simulink model "s_b4a4x1kf"  (R2018a)
settings: Solver=VariableStepDiscrete  StartTime=0.0  StopTime=1  RelTol=1e-3
undefined symbols (not defined in the file): fft_stages, n_bits_ants, n_bits_xengs
libraries: xbsIndex_r4 x22055, xbsReplacements_r4 x30, casper_library_misc x29, casper_library_scopes x15, xps_library x4
(part 29 of 227)

== system s_b4a4x1kf/sys1/vacc_tvg0 ==
  note: This counter increments by
      | one per accumulation.
      | Might be buggy; not tested.
  note: this TVG injects the same
      | number for vector_len.
      | Increments on vector edge.
      | (ramp over time)
  note: this TVG increments on
      | each valid input and resets
      | on vector_edge.
      | (ramp over channels).
  sync_in : Inport
  valid_in : Inport  Port=2
  data_in : Inport  Port=3
  time_in : Inport  Port=4
  acc_start_time : Inport  Port=5
  acc_len : Inport  Port=6
  Delay{,2..8} (8 alike) : xbsIndex_r4/Delay  rst=off  infoeditControl=Selection of Reset will increase slice count due to use of real FFs and instead of SRLs  en=off  latency=1  reg_retiming=on  dbl_ovrd=off  block_type=delay
      Delay settings: xl_area=[0, 0, 0, 0, 0, 0, 0]
      Delay2 settings: infoedit=Hardware notes: A delay line is a chain, each link of which is an SRL16 or SRL32 followed by a flip-flop.  xl_area=[0, 0, 0, 0, 0, 0, 0]
  Delay1 : xbsIndex_r4/Delay  rst=off  infoeditControl=Selection of Reset will increase slice count due to use of real FFs and instead of SRLs  en=off  latency=2  reg_retiming=on  dbl_ovrd=off  block_type=delay
      settings: infoedit=Hardware notes: A delay line is a chain, each link of which is an SRL16 or SRL32 followed by a flip-flop.  xl_area=[0, 0, 0, 0, 0, 0, 0]
  Delay9 : xbsIndex_r4/Delay  rst=off  infoeditControl=Selection of Reset will increase slice count due to use of real FFs and instead of SRLs  en=off  latency=3  reg_retiming=on  dbl_ovrd=off  block_type=delay
      settings: infoedit=Hardware notes: A delay line is a chain, each link of which is an SRL16 or SRL32 followed by a flip-flop.
  Mux1 : xbsIndex_r4/Mux  inputs=2  en=off  latency=1  precision=Full  arith_type="Signed  (2's comp)"  n_bits=8  bin_pt=2  quantization=Truncate  overflow=Wrap  dbl_ovrd=off  block_type=mux
      settings: xl_area=[0, 0, 0, 0, 0, 0, 0]
  Mux2 : xbsIndex_r4/Mux  inputs=2  en=off  latency=1  precision=Full  arith_type="Signed  (2's comp)"  n_bits=8  bin_pt=2  quantization=Truncate  overflow=Wrap  dbl_ovrd=off  block_type=mux
      settings: xl_area=[0, 0, 0, 0, 0, 0, 0]
  Mux3 : xbsIndex_r4/Mux  inputs=2  en=off  latency=1  precision=Full  arith_type="Signed  (2's comp)"  n_bits=8  bin_pt=2  quantization=Truncate  overflow=Wrap  dbl_ovrd=off  block_type=mux
      settings: xl_area=[0, 0, 0, 0, 0, 0, 0]
  Pulse Generator3 : DiscretePulseGenerator  Amplitude=25  Period=99999999  PulseWidth=500000  PhaseDelay=450000
  Relational2 : xbsIndex_r4/Relational  mode=a=b  op_type=Bool  en=off  latency=1  dbl_ovrd=off  block_type=relational
      settings: block_version=10.1.3
  Slice8 : xbsIndex_r4/Slice  nbits=n_bits  boolean_output=off  mode=Lower Bit Location + Width  bit1=0  base1=MSB of Input  bit0=0  base0=LSB of Input  dbl_ovrd=off  block_type=slice
  Slice9 : xbsIndex_r4/Slice  nbits=n_bits  boolean_output=off  mode=Lower Bit Location + Width  bit1=0  base1=MSB of Input  bit0=0  base0=LSB of Input  dbl_ovrd=off  block_type=slice
  Terminator5 : Terminator
  bus_replicate1 : Subsystem  Tag=cmac_delinked  mask(bus_replicate){replication=n_inputs, csp_latency=0, misc=off, implementation=core}
      mask prompts: replication "replication factor"; csp_latency "latency"; misc "misc support"; implementation "delay implementation"
      mask help: Output bus formed by replicating input bus a number of times
      mask init:
      | bus_replicate_init(gcb, ...
      |     'replication', replication, ...
      |     'csp_latency', csp_latency, ...
      |     'implementation', implementation, ...
      |     'misc', misc);
      mask TypeOptions implementation: core | behavioral
  bus_replicate2 : Subsystem  Tag=cmac_delinked  mask(bus_replicate){replication=n_inputs, csp_latency=0, misc=off, implementation=core}
      mask prompts: replication "replication factor"; csp_latency "latency"; misc "misc support"; implementation "delay implementation"
      mask help: Output bus formed by replicating input bus a number of times
      mask init:
      | bus_replicate_init(gcb, ...
      |     'replication', replication, ...
      |     'csp_latency', csp_latency, ...
      |     'implementation', implementation, ...
      |     'misc', misc);
      mask TypeOptions implementation: core | behavioral
  edge_detect : Subsystem  mask(edge_detect){edge=Rising, polarity=Active High, x_in=[0 0.08 0.08 0.16 0.16 0.24 0.24 0.32 0.32 0.4], y_in=[-1 -1  1  1  1  1  1  1  1  1], x_out=[0.6 0.68 0.68 0.76 0.76 0.84 0.84 0.92 0.92 1], y_out=[-1 -1  1  1 -1 -1 -1 -1 -1 -1]}
      mask prompts: edge "Edge Type"; polarity "Output Polarity"; x_in "Input X Positions"; y_in "Input Y Positions"; x_out "Output X Positions"; y_out "Output Y Positions"
      mask help: Output is active for one-cycle after each edge of the specified type (i.e. rising, falling or both).
      mask init: same as s_b4a4x1kf/edge_detect
      settings: AttributesFormatString=|
      | rising edges
      | active high
      mask Help: Output is active for one-cycle after each edge of the specified type (i.e. rising, falling, or both).  Latency is zero.
      mask TypeOptions edge: Rising | Falling | Both
      mask TypeOptions polarity: Active High | Active Low
      mask Display:
      | plot(x_in_num,0.5+y_in_num*0.2);
      | plot(x_out_num,0.5+y_out_num*0.2);
  edge_detect4 : Subsystem  mask(edge_detect){edge=Rising, polarity=Active High, x_in=[0 0.08 0.08 0.16 0.16 0.24 0.24 0.32 0.32 0.4], y_in=[-1 -1  1  1  1  1  1  1  1  1], x_out=[0.6 0.68 0.68 0.76 0.76 0.84 0.84 0.92 0.92 1], y_out=[-1 -1  1  1 -1 -1 -1 -1 -1 -1]}
      mask prompts: edge "Edge Type"; polarity "Output Polarity"; x_in "Input X Positions"; y_in "Input Y Positions"; x_out "Output X Positions"; y_out "Output Y Positions"
      mask help: Output is active for one-cycle after each edge of the specified type (i.e. rising, falling or both).
      mask init: same as s_b4a4x1kf/edge_detect
      settings: AttributesFormatString=|
      | rising edges
      | active high
      mask Help: Output is active for one-cycle after each edge of the specified type (i.e. rising, falling, or both).  Latency is zero.
      mask TypeOptions edge: Rising | Falling | Both
      mask TypeOptions polarity: Active High | Active Low
      mask Display:
      | plot(x_in_num,0.5+y_in_num*0.2);
      | plot(x_out_num,0.5+y_out_num*0.2);
  generate_pulses : Subsystem
  generate_time : Subsystem  mask{vec_len=len, n_inputs=n_inputs, n_bits=n_bits}
      mask prompts: vec_len "Vector Length?"; n_inputs "Simultaneous inputs"; n_bits "Data width"
      mask init:
      | vector_bits=ceil(log2(vec_len));
      | fmtstr = sprintf('Vector Length: %d', vec_len);
      | set_param(gcb, 'AttributesFormatString', fmtstr);
      settings: AttributesFormatString=Vector Length: 640
  group_period : Subsystem  Tag=xps:sw_reg  AncestorBlock=xps_library/Memory/software_register  mask(swreg){io_dir=From Processor, io_delay=0, init_val=0, sample_period=1, names=reg, bitwidths=32, bin_pts=0, arith_types=0, sim_port=on, show_format=on}
      mask prompts: io_dir "I/O direction"; io_delay "I/O delay"; init_val "Initial Value"; sample_period "Sample period"; names "Bitfield names [msb...lsb]"; bitwidths "Bitfield widths"; bin_pts "Bitfield binary pts"; arith_types "Bitfield types, ufix=0, fix=1, bool=2"; sim_port "Provide sim input/output?"; show_format "Print format string?"
      mask help: A 32-bit software-accessible register. Can be divided into bitfields of varying widths and types using the fields in the block mask.
      mask init:
      | swreg_init(gcb)
      settings: AttributesFormatString=1input:uf32.0 = 32 bits
      mask TypeOptions io_dir: To Processor | From Processor
      mask Callback io_dir:
      | mask_enables = get_param(gcb, 'MaskEnables');
      | mask_names = get_param(gcb, 'MaskNames');
      | if strcmp(get_param(gcb, 'io_dir'), 'To Processor'),
      |     mask_enables{ismember(mask_names, 'sample_period')} = 'off';
      | else
      |     mask_enables{ismember(mask_names, 'sample_period')} = 'on';
      | end
      | set_param(gcb, 'MaskEnables', mask_enables);
      mask DialogControl ParameterTabVar0 Prompt: Setup
  ins_counter : Subsystem  mask{vec_len=len, n_inputs=n_inputs, n_bits=n_bits}
      mask prompts: vec_len "Vector Length?"; n_inputs "Simultaneous inputs"; n_bits "Data width"
      mask init:
      | fmtstr = sprintf('Vector Length: %d', vec_len);
      | set_param(gcb, 'AttributesFormatString', fmtstr);
      settings: AttributesFormatString=Vector Length: 640
  ins_counter2 : Subsystem  mask{vec_len=len, n_inputs=n_inputs, n_bits=n_bits}
      mask prompts: vec_len "Vector Length?"; n_inputs "Simultaneous inputs"; n_bits "Data width"
      mask init:
      | vector_bits=ceil(log2(vec_len));
      | fmtstr = sprintf('Vector Length: %d', vec_len);
      | set_param(gcb, 'AttributesFormatString', fmtstr);
      settings: AttributesFormatString=Vector Length: 640
  ins_counter3 : Subsystem  mask{vec_len=len, n_inputs=n_inputs, n_bits=n_bits}
      mask prompts: vec_len "Vector Length?"; n_inputs "Simultaneous inputs"; n_bits "Data width"
      mask init:
      | vector_bits=ceil(log2(vec_len));
      | fmtstr = sprintf('Vector Length: %d', vec_len);
      | set_param(gcb, 'AttributesFormatString', fmtstr);
      settings: AttributesFormatString=Vector Length: 640
  ins_vect_loc : Subsystem  Tag=xps:sw_reg  AncestorBlock=xps_library/Memory/software_register  mask(swreg){io_dir=From Processor, io_delay=0, init_val=0, sample_period=1, names=reg, bitwidths=32, bin_pts=0, arith_types=0, sim_port=on, show_format=on}
      mask prompts: io_dir "I/O direction"; io_delay "I/O delay"; init_val "Initial Value"; sample_period "Sample period"; names "Bitfield names [msb...lsb]"; bitwidths "Bitfield widths"; bin_pts "Bitfield binary pts"; arith_types "Bitfield types, ufix=0, fix=1, bool=2"; sim_port "Provide sim input/output?"; show_format "Print format string?"
      mask help: A 32-bit software-accessible register. Can be divided into bitfields of varying widths and types using the fields in the block mask.
      mask init:
      | swreg_init(gcb)
      settings: AttributesFormatString=1input:uf32.0 = 32 bits
      mask TypeOptions io_dir: To Processor | From Processor
      mask Callback io_dir:
      | mask_enables = get_param(gcb, 'MaskEnables');
      | mask_names = get_param(gcb, 'MaskNames');
      | if strcmp(get_param(gcb, 'io_dir'), 'To Processor'),
      |     mask_enables{ismember(mask_names, 'sample_period')} = 'off';
      | else
      |     mask_enables{ismember(mask_names, 'sample_period')} = 'on';
      | end
      | set_param(gcb, 'MaskEnables', mask_enables);
      mask DialogControl ParameterTabVar0 Prompt: Setup
  ins_vect_val : Subsystem  Tag=xps:sw_reg  AncestorBlock=xps_library/Memory/software_register  mask(swreg){io_dir=From Processor, io_delay=0, init_val=0, sample_period=1, names=reg, bitwidths=32, bin_pts=0, arith_types=0, sim_port=on, show_format=on}
      mask prompts: io_dir "I/O direction"; io_delay "I/O delay"; init_val "Initial Value"; sample_period "Sample period"; names "Bitfield names [msb...lsb]"; bitwidths "Bitfield widths"; bin_pts "Bitfield binary pts"; arith_types "Bitfield types, ufix=0, fix=1, bool=2"; sim_port "Provide sim input/output?"; show_format "Print format string?"
      mask help: A 32-bit software-accessible register. Can be divided into bitfields of varying widths and types using the fields in the block mask.
      mask init:
      | swreg_init(gcb)
      settings: AttributesFormatString=1input:uf32.0 = 32 bits
      mask TypeOptions io_dir: To Processor | From Processor
      mask Callback io_dir:
      | mask_enables = get_param(gcb, 'MaskEnables');
      | mask_names = get_param(gcb, 'MaskNames');
      | if strcmp(get_param(gcb, 'io_dir'), 'To Processor'),
      |     mask_enables{ismember(mask_names, 'sample_period')} = 'off';
      | else
      |     mask_enables{ismember(mask_names, 'sample_period')} = 'on';
      | end
      | set_param(gcb, 'MaskEnables', mask_enables);
      mask DialogControl ParameterTabVar0 Prompt: Setup
  ins_vector : Subsystem  mask{num_vectors=len}
      mask prompts: num_vectors "number of vectors"
      mask init:
      | fmtstr = sprintf('Vector Length: %d', num_vectors);
      | set_param(gcb, 'AttributesFormatString', fmtstr);
      settings: AttributesFormatString=Vector Length: 640
  master_reset_sim1 : Constant
  master_reset_sim2 : Constant  Value=51200000
  master_reset_sim3 : Constant  Value=3
  master_reset_sim5 : Constant  Value=7
  master_reset_sim6 : Constant  Value=10
  master_reset_sim7 : Constant
  n_per_group : Subsystem  Tag=xps:sw_reg  AncestorBlock=xps_library/Memory/software_register  mask(swreg){io_dir=From Processor, io_delay=0, init_val=0, sample_period=1, names=reg, bitwidths=32, bin_pts=0, arith_types=0, sim_port=on, show_format=on}
      mask prompts: io_dir "I/O direction"; io_delay "I/O delay"; init_val "Initial Value"; sample_period "Sample period"; names "Bitfield names [msb...lsb]"; bitwidths "Bitfield widths"; bin_pts "Bitfield binary pts"; arith_types "Bitfield types, ufix=0, fix=1, bool=2"; sim_port "Provide sim input/output?"; show_format "Print format string?"
      mask help: A 32-bit software-accessible register. Can be divided into bitfields of varying widths and types using the fields in the block mask.
      mask init:
      | swreg_init(gcb)
      settings: AttributesFormatString=1input:uf32.0 = 32 bits
      mask TypeOptions io_dir: To Processor | From Processor
      mask Callback io_dir:
      | mask_enables = get_param(gcb, 'MaskEnables');
      | mask_names = get_param(gcb, 'MaskNames');
      | if strcmp(get_param(gcb, 'io_dir'), 'To Processor'),
      |     mask_enables{ismember(mask_names, 'sample_period')} = 'off';
      | else
      |     mask_enables{ismember(mask_names, 'sample_period')} = 'on';
      | end
      | set_param(gcb, 'MaskEnables', mask_enables);
      mask DialogControl ParameterTabVar0 Prompt: Setup
  n_pulses : Subsystem  Tag=xps:sw_reg  AncestorBlock=xps_library/Memory/software_register  mask(swreg){io_dir=From Processor, io_delay=0, init_val=0, sample_period=1, names=reg, bitwidths=32, bin_pts=0, arith_types=0, sim_port=on, show_format=on}
      mask prompts: io_dir "I/O direction"; io_delay "I/O delay"; init_val "Initial Value"; sample_period "Sample period"; names "Bitfield names [msb...lsb]"; bitwidths "Bitfield widths"; bin_pts "Bitfield binary pts"; arith_types "Bitfield types, ufix=0, fix=1, bool=2"; sim_port "Provide sim input/output?"; show_format "Print format string?"
      mask help: A 32-bit software-accessible register. Can be divided into bitfields of varying widths and types using the fields in the block mask.
      mask init:
      | swreg_init(gcb)
      settings: AttributesFormatString=1input:uf32.0 = 32 bits
      mask TypeOptions io_dir: To Processor | From Processor
      mask Callback io_dir:
      | mask_enables = get_param(gcb, 'MaskEnables');
      | mask_names = get_param(gcb, 'MaskNames');
      | if strcmp(get_param(gcb, 'io_dir'), 'To Processor'),
      |     mask_enables{ismember(mask_names, 'sample_period')} = 'off';
      | else
      |     mask_enables{ismember(mask_names, 'sample_period')} = 'on';
      | end
      | set_param(gcb, 'MaskEnables', mask_enables);
      mask DialogControl ParameterTabVar0 Prompt: Setup
  pipeline1 : Subsystem  mask(pipeline){csp_latency=3}
      mask prompts: csp_latency "Latency"
      mask help:
      | An explicitly laid-out delay line to avoid mapping to SRL16s
      | for use in pipelining to help achieve timing closure.
      mask init:
      | pipeline_init(gcb,'latency',csp_latency);
      settings: AttributesFormatString=Latency = %<latency>
      mask Display:
      | port_label('input', 1, 'd');
      | port_label('output', 1, 'q');
      | disp(['Z^-', num2str(csp_latency)]);
  pipeline2 : Subsystem  mask(pipeline){csp_latency=3}
      mask prompts: csp_latency "Latency"
      mask help:
      | An explicitly laid-out delay line to avoid mapping to SRL16s
      | for use in pipelining to help achieve timing closure.
      mask init:
      | pipeline_init(gcb,'latency',csp_latency);
      settings: AttributesFormatString=Latency = %<latency>
      mask Display:
      | port_label('input', 1, 'd');
      | port_label('output', 1, 'q');
      | disp(['Z^-', num2str(csp_latency)]);
  pipeline3 : Subsystem  mask(pipeline){csp_latency=3}
      mask prompts: csp_latency "Latency"
      mask help:
      | An explicitly laid-out delay line to avoid mapping to SRL16s
      | for use in pipelining to help achieve timing closure.
      mask init:
      | pipeline_init(gcb,'latency',csp_latency);
      settings: AttributesFormatString=Latency = %<latency>
      mask Display:
      | port_label('input', 1, 'd');
      | port_label('output', 1, 'q');
      | disp(['Z^-', num2str(csp_latency)]);
  pipeline4 : Subsystem  mask(pipeline){csp_latency=3}
      mask prompts: csp_latency "Latency"
      mask help:
      | An explicitly laid-out delay line to avoid mapping to SRL16s
      | for use in pipelining to help achieve timing closure.
      mask init:
      | pipeline_init(gcb,'latency',csp_latency);
      settings: AttributesFormatString=Latency = %<latency>
      mask Display:
      | port_label('input', 1, 'd');
      | port_label('output', 1, 'q');
      | disp(['Z^-', num2str(csp_latency)]);
  pipeline7 : Subsystem  mask(pipeline){csp_latency=3}
      mask prompts: csp_latency "Latency"
      mask help:
      | An explicitly laid-out delay line to avoid mapping to SRL16s
      | for use in pipelining to help achieve timing closure.
      mask init:
      | pipeline_init(gcb,'latency',csp_latency);
      settings: AttributesFormatString=Latency = %<latency>
      mask Display:
      | port_label('input', 1, 'd');
      | port_label('output', 1, 'q');
      | disp(['Z^-', num2str(csp_latency)]);
  ts_offset : Subsystem  Tag=xps:sw_reg  AncestorBlock=xps_library/Memory/software_register  mask(swreg){io_dir=From Processor, io_delay=0, init_val=0, sample_period=1, names=reg, bitwidths=32, bin_pts=0, arith_types=0, sim_port=on, show_format=off}
      mask prompts: io_dir "I/O direction"; io_delay "I/O delay"; init_val "Initial Value"; sample_period "Sample period"; names "Bitfield names [msb...lsb]"; bitwidths "Bitfield widths"; bin_pts "Bitfield binary pts"; arith_types "Bitfield types, ufix=0, fix=1, bool=2"; sim_port "Provide sim input/output?"; show_format "Print format string?"
      mask help: A 32-bit software-accessible register. Can be divided into bitfields of varying widths and types using the fields in the block mask.
      mask init:
      | swreg_init(gcb)
      settings: AttributesFormatString=1input
      mask TypeOptions io_dir: To Processor | From Processor
      mask Callback io_dir:
      | mask_enables = get_param(gcb, 'MaskEnables');
      | mask_names = get_param(gcb, 'MaskNames');
      | if strcmp(get_param(gcb, 'io_dir'), 'To Processor'),
      |     mask_enables{ismember(mask_names, 'sample_period')} = 'off';
      | else
      |     mask_enables{ismember(mask_names, 'sample_period')} = 'on';
      | end
      | set_param(gcb, 'MaskEnables', mask_enables);
      mask DialogControl ParameterTabVar0 Prompt: Setup
  write : Subsystem  Tag=xps:sw_reg  AncestorBlock=xps_library/Memory/software_register  mask(swreg){io_dir=From Processor, io_delay=0, init_val=0, sample_period=1, names=reg, bitwidths=32, bin_pts=0, arith_types=0, sim_port=on, show_format=on}
      mask prompts: io_dir "I/O direction"; io_delay "I/O delay"; init_val "Initial Value"; sample_period "Sample period"; names "Bitfield names [msb...lsb]"; bitwidths "Bitfield widths"; bin_pts "Bitfield binary pts"; arith_types "Bitfield types, ufix=0, fix=1, bool=2"; sim_port "Provide sim input/output?"; show_format "Print format string?"
      mask help: A 32-bit software-accessible register. Can be divided into bitfields of varying widths and types using the fields in the block mask.
      mask init:
      | swreg_init(gcb)
      settings: AttributesFormatString=1input:uf32.0 = 32 bits
      mask TypeOptions io_dir: To Processor | From Processor
      mask Callback io_dir:
      | mask_enables = get_param(gcb, 'MaskEnables');
      | mask_names = get_param(gcb, 'MaskNames');
      | if strcmp(get_param(gcb, 'io_dir'), 'To Processor'),
      |     mask_enables{ismember(mask_names, 'sample_period')} = 'off';
      | else
      |     mask_enables{ismember(mask_names, 'sample_period')} = 'on';
      | end
      | set_param(gcb, 'MaskEnables', mask_enables);
      mask DialogControl ParameterTabVar0 Prompt: Setup
  data_out : Outport
  valid_out : Outport  Port=2
  time_out : Outport  Port=3
  wires:
  pipeline2/1(q) -> generate_pulses/4(group period)
  pipeline1/1(q) -> generate_pulses/3(num_per_group)
  pipeline7/1(q) -> generate_pulses/2(num_pulses)
  Delay1/1 -> Mux1/3
  write/1(in_reg) -> Slice8/1
  master_reset_sim1/1 -> write/1(sim_1)
  [vacctvg_reset] -> Delay2/1
  valid_in/1 -> Mux1/2
  ins_vector/2(data) -> data_out/1
  ins_vector/3(valid_out) -> valid_out/1
  data_in/1 -> Mux2/2
  sync_in/1 -> Mux3/2
  [vacctvg_sync_sel] -> Mux3/1
  [vacctvg_data_sel] -> Mux2/1
  [vacctvg_valid_sel] -> Mux1/1
  [vacctvg_pulse_en] -> Delay/1
  generate_pulses/1(valid) -> Delay1/1
  edge_detect/1(out) -> Mux3/3
  [vacctvg_vector_en] -> ins_vector/6(enable)
  [vector_loc] -> ins_vector/4(vector)
  [vacctvg_ctr_en] -> ins_counter/4(enable)
  Delay/1 -> generate_pulses/1(run)
  generate_pulses/2(running) -> Terminator5/1
  [vector_val] -> ins_vector/5(value)
  Slice8/1 -> bus_replicate1/1(in)
  bus_replicate1/1(out) -> Mux2/3
  ins_vector/4(misco) -> time_out/1
  n_pulses/1(in_reg) -> pipeline7/1(d)
  n_per_group/1(in_reg) -> pipeline1/1(d)
  group_period/1(in_reg) -> pipeline2/1(d)
  master_reset_sim2/1 -> n_pulses/1(sim_1)
  master_reset_sim3/1 -> n_per_group/1(sim_1)
  master_reset_sim5/1 -> group_period/1(sim_1)
  master_reset_sim7/1 -> ins_vect_loc/1(sim_1)
  master_reset_sim6/1 -> ins_vect_val/1(sim_1)
  ins_vect_loc/1(in_reg) -> pipeline3/1(d)
  ins_vect_val/1(in_reg) -> pipeline4/1(d)
  Slice9/1 -> bus_replicate2/1(in)
  pipeline4/1(q) -> Slice9/1
  bus_replicate2/1(out) -> [vector_val]
  pipeline3/1(q) -> [vector_loc]
  Delay2/1 -> edge_detect/1(in)
  ins_counter/1(new_acc_out) -> ins_vector/1(new_acc_in)
  ins_counter/4(misco) -> ins_vector/7(misci)
  ins_counter/2(dout) -> ins_vector/2(data_in)
  ins_counter/3(valid_out) -> ins_vector/3(valid_in)
  ts_offset/1(in_reg) -> Delay8/1
  Pulse Generator3/1 -> ts_offset/1(sim_1)
  ins_counter2/2(dout) -> ins_counter/2(din)
  ins_counter2/3(valid_out) -> ins_counter/3(valid_in)
  ins_counter2/4(time_out) -> ins_counter/5(misci)
  [vacctvg_ctr2_en] -> ins_counter2/4(cnt_tvg_en)
  ins_counter2/1(sync_out) -> ins_counter/1(new_acc_in)
  time_in/1 -> Delay3/1
  Delay8/1 -> generate_time/6(offset)
  [vacctvg_time_sel] -> generate_time/4(time_tvg_en)
  Mux1/1 -> generate_time/3(valid_in)
  Mux2/1 -> generate_time/2(din)
  Mux3/1 -> generate_time/1(sync_in)
  Delay3/1 -> generate_time/5(time_in)
  edge_detect4/1(out) -> Delay9/1, ins_counter3/6(cnt_rst)
  generate_time/1(sync_out) -> Delay7/1
  generate_time/2(dout) -> Delay6/1
  generate_time/3(valid_out) -> Delay5/1
  ins_counter3/1(sync_out) -> ins_counter2/1(sync_in)
  ins_counter3/2(dout) -> ins_counter2/2(din)
  ins_counter3/3(valid_out) -> ins_counter2/3(valid_in)
  ins_counter3/4(time_out) -> ins_counter2/5(time_in)
  [vacctvg_ctr3_en] -> ins_counter3/4(cnt_tvg_en)
  acc_len/1 -> ins_counter3/7(acc_len)
  Relational2/1 -> edge_detect4/1(in)
  acc_start_time/1 -> Relational2/2
  generate_time/4(time_out) -> Relational2/1, Delay4/1
  Delay4/1 -> ins_counter3/5(time_in)
  Delay5/1 -> ins_counter3/3(valid_in)
  Delay6/1 -> ins_counter3/2(din)
  Delay7/1 -> ins_counter3/1(sync_in)
  Delay9/1 -> ins_counter2/6(cnt_rst)

== system s_b4a4x1kf/sys1/x_cast ==
  in : Inport
  Concat : xbsIndex_r4/Concat  num_inputs=8  dbl_ovrd=off  block_type=concat
      settings: block_version=9.2.01
  Convert{,1..7} (8 alike) : xbsIndex_r4/Convert  gui_display_data_type=Fixed-point  arith_type="Signed  (2's comp)"  n_bits=n_bits_out  bin_pt=fix_pnt_pos  float_type=Single  exp_bits=8  fraction_bits=24  quantization=Truncate  overflow=Wrap  en=off  latency=0  pipeline=off  dbl_ovrd=off  block_type=convert
      settings: block_version=10.1.3
  Slice : xbsIndex_r4/Slice  nbits=n_bits_in  boolean_output=off  mode=Lower Bit Location + Width  bit1=0  base1=MSB of Input  bit0=bit_offsets(1)*n_bits_in  base0=LSB of Input  dbl_ovrd=off  block_type=slice
      settings: infoedit="Extracts a given range of bits from each input sample and presents it at the output.  The output type is ordinarily unsigned with binary point at zero, but can be Boolean when the slice is one bit wide.<P><P>Hardware notes: In hardware this block costs nothing."  block_version=10.1.3
  Slice1 : xbsIndex_r4/Slice  nbits=n_bits_in  boolean_output=off  mode=Lower Bit Location + Width  bit1=0  base1=MSB of Input  bit0=bit_offsets(2)*n_bits_in  base0=LSB of Input  dbl_ovrd=off  block_type=slice
      settings: infoedit="Extracts a given range of bits from each input sample and presents it at the output.  The output type is ordinarily unsigned with binary point at zero, but can be Boolean when the slice is one bit wide.<P><P>Hardware notes: In hardware this block costs nothing."  block_version=10.1.3
  Slice2 : xbsIndex_r4/Slice  nbits=n_bits_in  boolean_output=off  mode=Lower Bit Location + Width  bit1=0  base1=MSB of Input  bit0=bit_offsets(3)*n_bits_in  base0=LSB of Input  dbl_ovrd=off  block_type=slice
      settings: infoedit="Extracts a given range of bits from each input sample and presents it at the output.  The output type is ordinarily unsigned with binary point at zero, but can be Boolean when the slice is one bit wide.<P><P>Hardware notes: In hardware this block costs nothing."  block_version=10.1.3
  Slice3 : xbsIndex_r4/Slice  nbits=n_bits_in  boolean_output=off  mode=Lower Bit Location + Width  bit1=0  base1=MSB of Input  bit0=bit_offsets(4)*n_bits_in  base0=LSB of Input  dbl_ovrd=off  block_type=slice
      settings: infoedit="Extracts a given range of bits from each input sample and presents it at the output.  The output type is ordinarily unsigned with binary point at zero, but can be Boolean when the slice is one bit wide.<P><P>Hardware notes: In hardware this block costs nothing."  block_version=10.1.3
  Slice4 : xbsIndex_r4/Slice  nbits=n_bits_in  boolean_output=off  mode=Lower Bit Location + Width  bit1=0  base1=MSB of Input  bit0=bit_offsets(5)*n_bits_in  base0=LSB of Input  dbl_ovrd=off  block_type=slice
      settings: infoedit="Extracts a given range of bits from each input sample and presents it at the output.  The output type is ordinarily unsigned with binary point at zero, but can be Boolean when the slice is one bit wide.<P><P>Hardware notes: In hardware this block costs nothing."  block_version=10.1.3
  Slice5 : xbsIndex_r4/Slice  nbits=n_bits_in  boolean_output=off  mode=Lower Bit Location + Width  bit1=0  base1=MSB of Input  bit0=bit_offsets(6)*n_bits_in  base0=LSB of Input  dbl_ovrd=off  block_type=slice
      settings: infoedit="Extracts a given range of bits from each input sample and presents it at the output.  The output type is ordinarily unsigned with binary point at zero, but can be Boolean when the slice is one bit wide.<P><P>Hardware notes: In hardware this block costs nothing."  block_version=10.1.3
  Slice6 : xbsIndex_r4/Slice  nbits=n_bits_in  boolean_output=off  mode=Lower Bit Location + Width  bit1=0  base1=MSB of Input  bit0=bit_offsets(7)*n_bits_in  base0=LSB of Input  dbl_ovrd=off  block_type=slice
      settings: infoedit="Extracts a given range of bits from each input sample and presents it at the output.  The output type is ordinarily unsigned with binary point at zero, but can be Boolean when the slice is one bit wide.<P><P>Hardware notes: In hardware this block costs nothing."  block_version=10.1.3
  Slice7 : xbsIndex_r4/Slice  nbits=n_bits_in  boolean_output=off  mode=Lower Bit Location + Width  bit1=0  base1=MSB of Input  bit0=bit_offsets(8)*n_bits_in  base0=LSB of Input  dbl_ovrd=off  block_type=slice
      settings: infoedit="Extracts a given range of bits from each input sample and presents it at the output.  The output type is ordinarily unsigned with binary point at zero, but can be Boolean when the slice is one bit wide.<P><P>Hardware notes: In hardware this block costs nothing."  block_version=10.1.3
  force_re{,1,4,6,8,10,12,14} (8 alike) : xbsIndex_r4/Reinterpret  force_arith_type=on  arith_type="Signed  (2's comp)"  force_bin_pt=on  bin_pt=fix_pnt_pos  block_type=reinterpret
      settings: infoedit="Changes signal type without altering the binary representation.   You can changed the signal between signed and unsigned, and relocate the binary point.<P><P>Hardware notes: In hardware this block costs nothing.<P><P>Example:  Suppose the input is 6 bits wide, signed, with 2 fractional bits, and the output is forced to unsigned with 0 fractional bits.  Then an input of -2.0 (1110.00 in binary 2's complement) becomes an output of 56 (111000 in binary)."  block_version=9.1.01
  force_re{2..3,5,7,9,11,13,15} (8 alike) : xbsIndex_r4/Reinterpret  force_arith_type=on  arith_type=Unsigned  force_bin_pt=on  bin_pt=0  block_type=reinterpret
      settings: infoedit="Changes signal type without altering the binary representation.   You can changed the signal between signed and unsigned, and relocate the binary point.<P><P>Hardware notes: In hardware this block costs nothing.<P><P>Example:  Suppose the input is 6 bits wide, signed, with 2 fractional bits, and the output is forced to unsigned with 0 fractional bits.  Then an input of -2.0 (1110.00 in binary 2's complement) becomes an output of 56 (111000 in binary)."  block_version=9.1.01
  out : Outport
  wires:
  force_re2/1 -> Concat/1
  Convert/1 -> force_re2/1
  Convert1/1 -> force_re3/1
  force_re/1 -> Convert/1
  force_re1/1 -> Convert1/1
  Slice/1 -> force_re/1
  in/1 -> Slice/1, Slice6/1, Slice7/1, Slice5/1, Slice4/1, Slice3/1, Slice2/1, Slice1/1
  Concat/1 -> out/1
  Slice1/1 -> force_re1/1
  force_re3/1 -> Concat/2
  Convert2/1 -> force_re5/1
  force_re4/1 -> Convert2/1
  Slice2/1 -> force_re4/1
  Convert3/1 -> force_re7/1
  force_re6/1 -> Convert3/1
  Slice3/1 -> force_re6/1
  Convert4/1 -> force_re9/1
  force_re8/1 -> Convert4/1
  Slice4/1 -> force_re8/1
  Convert5/1 -> force_re11/1
  force_re10/1 -> Convert5/1
  Slice5/1 -> force_re10/1
  Convert6/1 -> force_re13/1
  force_re12/1 -> Convert6/1
  Slice6/1 -> force_re12/1
  Convert7/1 -> force_re15/1
  force_re14/1 -> Convert7/1
  Slice7/1 -> force_re14/1
  force_re5/1 -> Concat/3
  force_re7/1 -> Concat/4
  force_re9/1 -> Concat/5
  force_re11/1 -> Concat/6
  force_re13/1 -> Concat/7
  force_re15/1 -> Concat/8

== system s_b4a4x1kf/sys1/xeng ==
  sync_in : Inport
  ant : Inport  Port=2
  window_valid : Inport  Port=3
  mcnt_in : Inport  Port=4
  Constant : xbsIndex_r4/Constant  const=0  gui_display_data_type=Fixed-point  arith_type=Unsigned  n_bits=200  bin_pt=14  preci_type=Single  exp_width=8  frac_width=24  explicit_period=on  period=1  equ=P=C  opselect=C  inp2=PCIN>>17  opr=+  inp1=P  carry=CIN  dbl_ovrd=off  block_type=constant
  Constant1 : xbsIndex_r4/Constant  const=0  gui_display_data_type=Fixed-point  arith_type=Boolean  n_bits=1  bin_pt=14  preci_type=Single  exp_width=8  frac_width=24  explicit_period=on  period=1  equ=P=C  opselect=C  inp2=PCIN>>17  opr=+  inp1=P  carry=CIN  dbl_ovrd=off  block_type=constant
  Term1 : Terminator
  Term2 : Terminator
  Term3 : Terminator
  auto_tap : Subsystem  mask(auto_tap){n_ants=4, n_simultan=2, n_bits=8, acc_len=256, add_latency=3, mult_latency=4, bram_latency=7, mult_type=1, use_bram_delay=1}
      mask prompts: n_ants "Number of antennas (total inputs = n_ants*n_simultan below)"; n_simultan "Number of inputs fed-in simultaneously"; n_bits "Number of input bits (per complex component)"; acc_len "Accumulation length"; add_latency "Adder latency"; mult_latency "Multiplier latency"; bram_latency "BRAM latency"; mult_type "Multiplier Type (0=behavioural HDL, 1=embedded, 2=core)"; use_bram_delay "Implementation: Delay type (0=SLR, 1=BRAM)"
      mask init:
      | fix_pnt_pos = (n_bits-1)*2;
      | bit_growth = ceil(log2(acc_len));
      | ant_bits = ceil(log2(n_ants));
      | n_bits_out = (2*n_bits + 1 + bit_growth);
      | 
      | params = get_mask_params(gcb);
      | auto_tap_init(gcb, params{:});
      settings: AttributesFormatString=mult_typ=1, del_typ=1
  baseline_tap1 : Subsystem  mask(baseline_tap){n_ants=4, ant_sep=1, n_bits=8, acc_len=256, add_latency=3, mult_latency=4, bram_latency=7, mult_type=1, use_bram_delay=1}
      mask prompts: n_ants "Number of antennas"; ant_sep "Antenna Seperation"; n_bits "number of input bits (per complex component)"; acc_len "accumulation length"; add_latency "Adder latency"; mult_latency "Multiplier latency"; bram_latency "BRAM latency"; mult_type "Multiplier Type (0=behavioural HDL, 1=embedded, 2=core)"; use_bram_delay "Use BRAM delays"
      mask init: same as s_b4a4x1kf/sys0/xeng/baseline_tap1
      settings: AttributesFormatString=ant_sep=1, mult=1, bram=1
  baseline_tap2 : Subsystem  mask(baseline_tap){n_ants=4, ant_sep=2, n_bits=8, acc_len=256, add_latency=3, mult_latency=4, bram_latency=7, mult_type=1, use_bram_delay=1}
      mask prompts: n_ants "Number of antennas"; ant_sep "Antenna Seperation"; n_bits "number of input bits (per complex component)"; acc_len "accumulation length"; add_latency "Adder latency"; mult_latency "Multiplier latency"; bram_latency "BRAM latency"; mult_type "Multiplier Type (0=behavioural HDL, 1=embedded, 2=core)"; use_bram_delay "Use BRAM delays"
      mask init: same as s_b4a4x1kf/sys0/xeng/baseline_tap1
      settings: AttributesFormatString=ant_sep=2, mult=1, bram=1
  delay : xbsIndex_r4/Delay  rst=off  infoeditControl=Selection of Reset will increase slice count due to use of real FFs and instead of SRLs  en=off  latency=1  reg_retiming=on  dbl_ovrd=off  block_type=delay
  sample_and_hold1 : Subsystem  mask(sample_and_hold){period=1024}
      mask prompts: period "Sample period (clocks)"
      mask help: This block will sample an input signal at a user specified rate and hold the value on the output.
  sample_and_hold2 : Subsystem  mask(sample_and_hold){period=1024}
      mask prompts: period "Sample period (clocks)"
      mask help: This block will sample an input signal at a user specified rate and hold the value on the output.
  sample_and_hold3 : Subsystem  mask(sample_and_hold){period=1024}
      mask prompts: period "Sample period (clocks)"
      mask help: This block will sample an input signal at a user specified rate and hold the value on the output.
  window_delay : Subsystem  mask{delay=267}
      mask prompts: delay "desired delay (>2)"
      mask Display: fprintf('Z^-%d', delay)
  xeng_descramble_4ant : Subsystem  mask(xeng_descramble){n_bits=8, acc_len=256, demux_factor=1}
      mask prompts: n_bits "Input Bitwidth"; acc_len "X engine accumulation length"; demux_factor "Demux Factor"
      mask help:
      | NOT TESTED FOR non-2^N antennas.
      |
      | Descrambles X engine output. Optionally demuxes output.
      mask init: same as s_b4a4x1kf/sys0/xeng/xeng_descramble_4ant
      settings: AttributesFormatString=num_ants=4
  sync_out : Outport
  valid : Outport  Port=2
  acc : Outport  Port=3
  mcnt_out : Outport  Port=4
  wires:
  baseline_tap2/4(acc_out) -> xeng_descramble_4ant/1(acc)
  baseline_tap2/5(valid_out) -> xeng_descramble_4ant/2(valid)
  baseline_tap2/7(sync_out) -> xeng_descramble_4ant/3(sync), sample_and_hold2/1(sync)
  window_delay/1(out) -> xeng_descramble_4ant/4(win_valid)
  xeng_descramble_4ant/1(acc_out) -> acc/1
  xeng_descramble_4ant/2(valid_out) -> valid/1
  xeng_descramble_4ant/3(sync_out) -> sync_out/1, sample_and_hold3/1(sync)
  ant/1 -> auto_tap/1(a_del), auto_tap/2(a_ndel)
  Constant/1 -> auto_tap/4(acc_in)
  Constant1/1 -> auto_tap/5(valid_in)
  sync_in/1 -> auto_tap/6(sync_in), sample_and_hold1/1(sync)
  window_valid/1 -> window_delay/1(in)
  mcnt_in/1 -> sample_and_hold1/2(in)
  sample_and_hold1/1(out) -> sample_and_hold2/2(in)
  sample_and_hold2/1(out) -> sample_and_hold3/2(in)
  sample_and_hold3/1(out) -> delay/1
  delay/1 -> mcnt_out/1
  auto_tap/1(a_del_out) -> baseline_tap1/1(a_del)
  auto_tap/2(a_ndel_out) -> baseline_tap1/2(a_ndel)
  auto_tap/3(a_end_out) -> baseline_tap1/3(a_end)
  auto_tap/4(acc_out) -> baseline_tap1/4(acc_in)
  auto_tap/5(valid_out) -> baseline_tap1/5(valid_in)
  auto_tap/6(rst_out) -> baseline_tap1/6(rst)
  auto_tap/7(sync_out) -> baseline_tap1/7(sync1)
  baseline_tap1/1(a_del_out) -> baseline_tap2/1(a_del)
  baseline_tap1/2(a_ndel_out) -> baseline_tap2/2(a_ndel)
  baseline_tap1/3(a_end_out) -> baseline_tap2/3(a_end)
  baseline_tap1/4(acc_out) -> baseline_tap2/4(acc_in)
  baseline_tap1/5(valid_out) -> baseline_tap2/5(valid_in)
  baseline_tap1/6(rst_out) -> baseline_tap2/6(rst)
  baseline_tap1/7(sync_out) -> baseline_tap2/7(sync1)
  baseline_tap2/1(a_del_out) -> auto_tap/3(a_loop)
  baseline_tap2/2(a_ndel_out) -> Term1/1
  baseline_tap2/3(a_end_out) -> Term2/1
  baseline_tap2/6(rst_out) -> Term3/1
